simulink model "L2"  (R2026b)
settings: Solver=VariableStepAuto
settings Model: Creator=Leonid  LastModifiedBy=Leonid

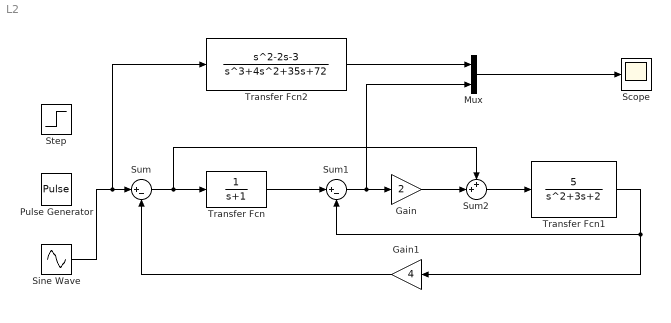
== system L2 ==
  Gain : Gain  Gain=2
  Gain1 : Gain  Gain=4
  Mux : Mux  Inputs=2
  Pulse Generator : DiscretePulseGenerator  PulseType=Time based  Period=10  PulseWidth=5
  Scope : Scope
      settings: ActiveDisplayYMinimum=-5.0951938116867712  ActiveDisplayYMaximum=2.3351932706532303
  Sine Wave : Sin  SampleTime=0
  Step : Step  SampleTime=0
  Sum : Sum  Inputs=|+-
  Sum1 : Sum  Inputs=|+-
  Sum2 : Sum  Inputs=++|
  Transfer Fcn : TransferFcn  Denominator=[1 1]
  Transfer Fcn1 : TransferFcn  Numerator=[5]  Denominator=[1 3 2]
  Transfer Fcn2 : TransferFcn  Numerator=[1 -2 -3]  Denominator=[1 4 35 72]
  wires:
  Sum/1 -> Sum2/1, Transfer Fcn/1
  Transfer Fcn/1 -> Sum1/1
  Gain/1 -> Sum2/2
  Gain1/1 -> Sum/2
  Sum1/1 -> Mux/2, Gain/1
  Sum2/1 -> Transfer Fcn1/1
  Transfer Fcn1/1 -> Sum1/2, Gain1/1
  Mux/1 -> Scope/1
  Transfer Fcn2/1 -> Mux/1
  Sine Wave/1 -> Transfer Fcn2/1, Sum/1
